simulink model "EBDsimu"  (R2024b)
settings: Solver=VariableStepAuto  StartTime=0.0  StopTime=10  RelTol=1e-3
values from neighbouring files (symbols this model uses):
  dar = 1.5    [EBD.m]
  dav = 1.5    [EBD.m]
  Flim = f*m*g/4    (= 1962)    [ABS.m]    (also in EBD.m)
  g = 9.81    [ABS.m]    (also in EBD.m)
  h = 0.7    [EBD.m]
  J = 0.5    [ABS.m]    (also in EBD.m; TD1_2_3.m = 0.2)
  Kd = 0    [ABS.m]    (also in EBD.m)
  Ki = 20    [ABS.m]    (also in EBD.m = 0)
  Kp = 50    [ABS.m]    (also in EBD.m = 1; TD1_2_3.m = 20)
  L = 3    [EBD.m]    (also in TD1_2_3.m = 0.01216)
  m = 1000    [ABS.m]    (also in EBD.m)
  rRoue = 0.3    [ABS.m]    (also in EBD.m)
  v0 = 27.77    [ABS.m]    (also in EBD.m)
  w0 = v0/rRoue    (= 92.5666666667)    [ABS.m]    (also in EBD.m)
undefined symbols (not defined in the file or in its folder): DiscIntNeverNeededParam
libraries: simulink x9
settings Model: Creator=E306-PC2  LastModifiedBy=clave

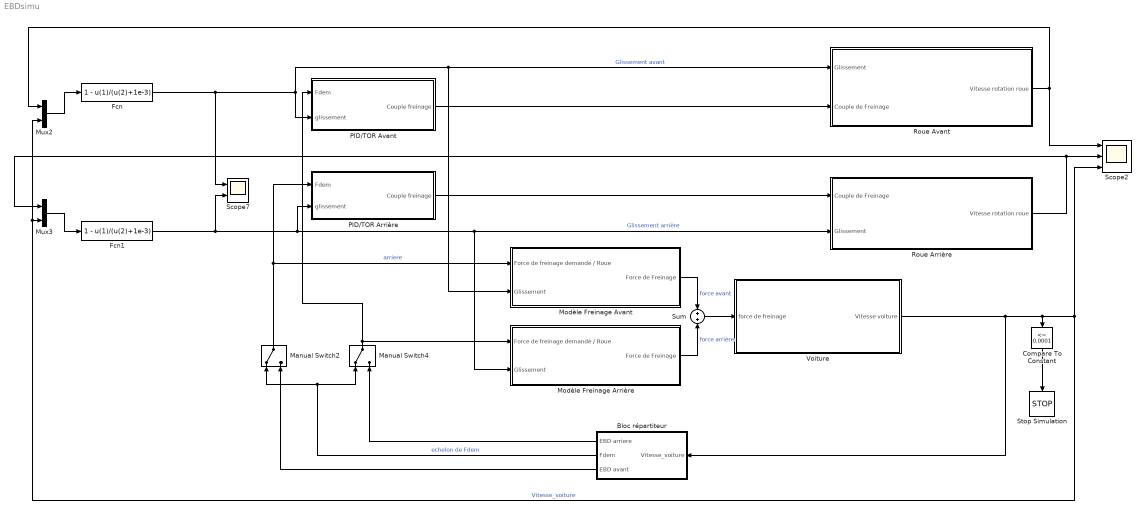
== system EBDsimu ==
  Bloc répartiteur : Subsystem
  Compare To Constant : simulink/Logic and Bit Operations/Compare To Constant  relop=<=  const=0.0001  OutDataTypeStr=boolean
  Fcn : Fcn  Expr=1 - u(1)/(u(2)+1e-3)
  Fcn1 : Fcn  Expr=1 - u(1)/(u(2)+1e-3)
  Manual Switch2 : ManualSwitch
  Manual Switch4 : ManualSwitch
  Modèle Freinage Arrière : Subsystem
  Modèle Freinage Avant : Subsystem
  Mux2 : Mux  Inputs=2
  Mux3 : Mux  Inputs=2
  PID/TOR Arrière : Subsystem
  PID/TOR Avant : Subsystem
  Roue Arrière : Subsystem
  Roue Avant : Subsystem
  Scope2 : Scope  NumInputPorts=3
  Scope7 : Scope  NumInputPorts=2
  Stop Simulation : Stop
  Sum : Sum
  Voiture : Subsystem
  wires:
  Roue Avant/1(Vitesse rotation roue) -> Scope2/1, Mux2/1
  Fcn/1 -> PID/TOR Avant/2(glissement), Roue Avant/1(Glissement), Modèle Freinage Avant/2(Glissement), Scope7/1  "Glissement avant"
  Roue Arrière/1(Vitesse rotation roue) -> Mux3/1, Scope2/2
  Fcn1/1 -> Scope7/2, Modèle Freinage Arrière/2(Glissement), Roue Arrière/2(Glissement), PID/TOR Arrière/2(glissement)  "Glissement arrière"
  Sum/1 -> Voiture/1(force de freinage)
  Mux2/1 -> Fcn/1
  Mux3/1 -> Fcn1/1
  Manual Switch2/1 -> PID/TOR Arrière/1(Fdem), Modèle Freinage Avant/1(Force de freinage demandé / Roue)  "arriere"
  Manual Switch4/1 -> PID/TOR Avant/1(Fdem), Modèle Freinage Arrière/1(Force de freinage demandé / Roue)
  Compare To Constant/1 -> Stop Simulation/1
  Voiture/1(Vitesse voiture) -> Bloc répartiteur/1(Vitesse_voiture), Compare To Constant/1, Scope2/3, Mux2/2, Mux3/2  "Vitesse_voiture"
  PID/TOR Arrière/1(Couple freinage) -> Roue Arrière/1(Couple de Freinage)
  PID/TOR Avant/1(Couple freinage) -> Roue Avant/2(Couple de Freinage)
  Modèle Freinage Avant/1(Force de Freinage) -> Sum/1  "force avant"
  Modèle Freinage Arrière/1(Force de Freinage) -> Sum/2  "force arrière"
  Bloc répartiteur/2(Fdem) -> Manual Switch2/1, Manual Switch4/1  "echelon de Fdem"
  Bloc répartiteur/3(EBD avant) -> Manual Switch2/2
  Bloc répartiteur/1(EBD arriere) -> Manual Switch4/2

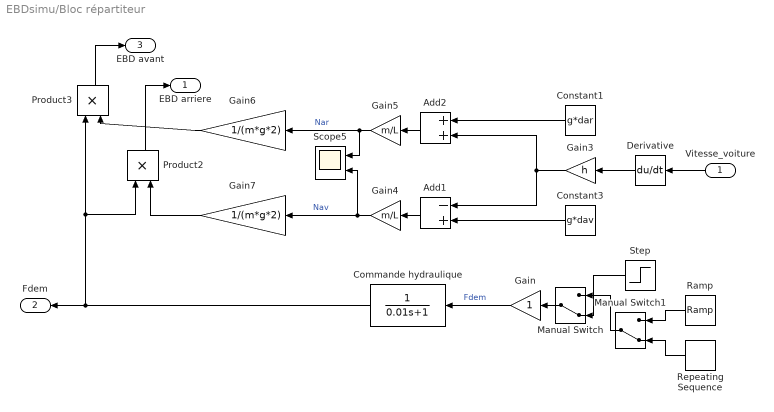
== system EBDsimu/Bloc répartiteur ==
  Vitesse_voiture : Inport
  Add1 : Sum  Inputs=-+
  Add2 : Sum
  Commande hydraulique : TransferFcn  Denominator=[0.01 1]
  Constant1 : Constant  Value=g*dar
  Constant3 : Constant  Value=g*dav
  Derivative : Derivative
  Gain : Gain
  Gain3 : Gain  Gain=h
  Gain4 : Gain  Gain=m/L
  Gain5 : Gain  Gain=m/L
  Gain6 : Gain  Gain=1/(m*g*2)
  Gain7 : Gain  Gain=1/(m*g*2)
  Manual Switch : ManualSwitch  CurrentSetting=0
  Manual Switch1 : ManualSwitch  CurrentSetting=0
  Product2 : Product
  Product3 : Product
  Ramp : simulink/Sources/Ramp  slope=4000  start=0  InitialOutput=0
  Repeating Sequence : simulink/Sources/Repeating Sequence  rep_seq_t=[0 0.5 3 3.5 10]  rep_seq_y=[0 5000 5000 0 0]
  Scope5 : Scope  NumInputPorts=2
  Step : Step  Time=0  After=5000  SampleTime=0
  EBD arriere : Outport
  Fdem : Outport  Port=2
  EBD avant : Outport  Port=3
  wires:
  Repeating Sequence/1 -> Manual Switch1/2
  Add2/1 -> Gain5/1
  Gain4/1 -> Scope5/2, Gain7/1  "Nav"
  Manual Switch1/1 -> Manual Switch/1
  Commande hydraulique/1 -> Fdem/1, Product3/1, Product2/1
  Manual Switch/1 -> Gain/1
  Derivative/1 -> Gain3/1
  Gain3/1 -> Add1/1, Add2/2
  Constant1/1 -> Add2/1
  Gain/1 -> Commande hydraulique/1  "Fdem"
  Gain7/1 -> Product2/2
  Product3/1 -> EBD avant/1
  Add1/1 -> Gain4/1
  Constant3/1 -> Add1/2
  Gain6/1 -> Product3/2
  Product2/1 -> EBD arriere/1
  Gain5/1 -> Scope5/1, Gain6/1  "Nar"
  Step/1 -> Manual Switch/2
  Ramp/1 -> Manual Switch1/1
  Vitesse_voiture/1 -> Derivative/1

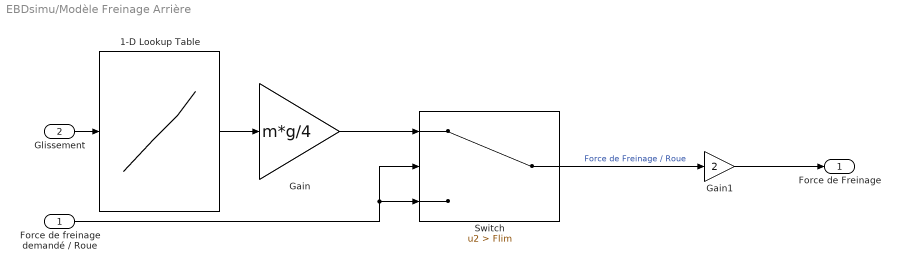
== system EBDsimu/Modèle Freinage Arrière ==
  Force de freinage demandé / Roue : Inport
  Glissement : Inport  Port=2
  1-D Lookup Table : Lookup_n-D  NumberOfTableDimensions=1  BreakpointsForDimension1=[0, 0.1, 0.2, 0.4, 0.6, 0.8, 1]  Table=[0, 0.85, 0.95, 0.75, 0.68, 0.63, 0.6]  InternalRulePriority=Speed  RndMeth=Simplest
  Gain : Gain  Gain=m*g/4
  Gain1 : Gain  Gain=2
  Switch : Switch  Criteria=u2 > Threshold  Threshold=Flim  SaturateOnIntegerOverflow=off  InputSameDT=off
  Force de Freinage : Outport
  wires:
  Gain/1 -> Switch/1
  Force de freinage demandé / Roue/1 -> Switch/3, Switch/2
  Glissement/1 -> 1-D Lookup Table/1
  Switch/1 -> Gain1/1  "Force de Freinage / Roue"
  1-D Lookup Table/1 -> Gain/1
  Gain1/1 -> Force de Freinage/1

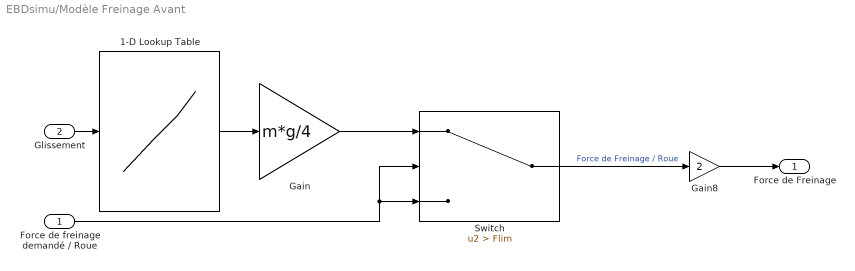
== system EBDsimu/Modèle Freinage Avant ==
  Force de freinage demandé / Roue : Inport
  Glissement : Inport  Port=2
  1-D Lookup Table : Lookup_n-D  NumberOfTableDimensions=1  BreakpointsForDimension1=[0, 0.1, 0.2, 0.4, 0.6, 0.8, 1]  Table=[0, 0.85, 0.95, 0.75, 0.68, 0.63, 0.6]  InternalRulePriority=Speed  RndMeth=Simplest
  Gain : Gain  Gain=m*g/4
  Gain8 : Gain  Gain=2
  Switch : Switch  Criteria=u2 > Threshold  Threshold=Flim  SaturateOnIntegerOverflow=off  InputSameDT=off
  Force de Freinage : Outport
  wires:
  Gain/1 -> Switch/1
  Force de freinage demandé / Roue/1 -> Switch/3, Switch/2
  Glissement/1 -> 1-D Lookup Table/1
  Switch/1 -> Gain8/1  "Force de Freinage / Roue"
  1-D Lookup Table/1 -> Gain/1
  Gain8/1 -> Force de Freinage/1

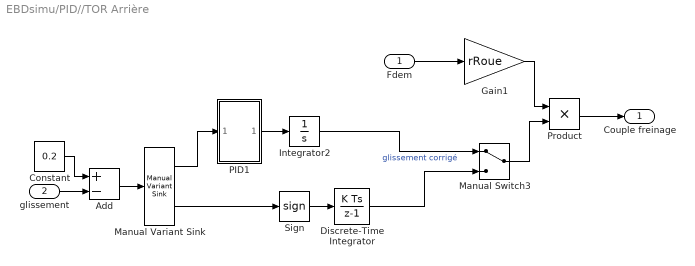
== system EBDsimu/PID//TOR Arrière ==
  Fdem : Inport
  glissement : Inport  Port=2
  Add : Sum  Inputs=+-
  Constant : Constant  Value=0.2
  Discrete-Time Integrator : DiscreteIntegrator  gainval=40  SampleTime=1e-4  LimitOutput=on  UpperSaturationLimit=Flim  ICPrevOutput=DiscIntNeverNeededParam  ICPrevScaledInput=DiscIntNeverNeededParam
  Gain1 : Gain  Gain=rRoue
  Integrator2 : Integrator  LimitOutput=on  UpperSaturationLimit=2000  LowerSaturationLimit=0
  Manual Variant Sink : simulink/Signal Routing/Manual Variant Sink  NumChoices=2  LabelModeActiveChoice=V_1
  Manual Switch3 : ManualSwitch
  PID1 : Subsystem
  Product : Product
  Sign : Signum
  Couple freinage : Outport
  wires:
  Gain1/1 -> Product/1
  Manual Switch3/1 -> Product/2
  Constant/1 -> Add/1
  Add/1 -> Manual Variant Sink/1
  Product/1 -> Couple freinage/1
  Fdem/1 -> Gain1/1
  glissement/1 -> Add/2
  Manual Variant Sink/2 -> Sign/1
  Sign/1 -> Discrete-Time Integrator/1
  Manual Variant Sink/1 -> PID1/1(1)
  Integrator2/1 -> Manual Switch3/1  "glissement corrigé"
  PID1/1(Out1) -> Integrator2/1
  Discrete-Time Integrator/1 -> Manual Switch3/2

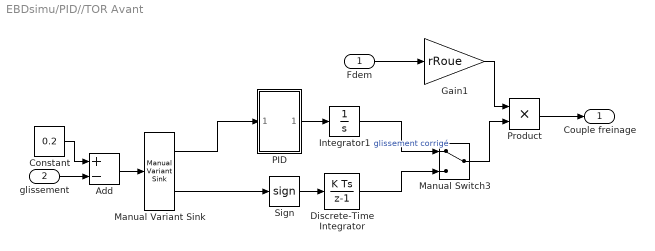
== system EBDsimu/PID//TOR Avant ==
  Fdem : Inport
  glissement : Inport  Port=2
  Add : Sum  Inputs=+-
  Constant : Constant  Value=0.2
  Discrete-Time Integrator : DiscreteIntegrator  gainval=40  SampleTime=1e-4  LimitOutput=on  UpperSaturationLimit=Flim  ICPrevOutput=DiscIntNeverNeededParam  ICPrevScaledInput=DiscIntNeverNeededParam
  Gain1 : Gain  Gain=rRoue
  Integrator1 : Integrator  LimitOutput=on  UpperSaturationLimit=2000  LowerSaturationLimit=0
  Manual Variant Sink : simulink/Signal Routing/Manual Variant Sink  NumChoices=2  LabelModeActiveChoice=V_1
  Manual Switch3 : ManualSwitch
  PID : Subsystem
  Product : Product
  Sign : Signum
  Couple freinage : Outport
  wires:
  Discrete-Time Integrator/1 -> Manual Switch3/2
  Gain1/1 -> Product/1
  Integrator1/1 -> Manual Switch3/1  "glissement corrigé"
  PID/1(Out1) -> Integrator1/1
  Manual Switch3/1 -> Product/2
  Constant/1 -> Add/1
  Product/1 -> Couple freinage/1
  Fdem/1 -> Gain1/1
  glissement/1 -> Add/2
  Manual Variant Sink/2 -> Sign/1
  Sign/1 -> Discrete-Time Integrator/1
  Add/1 -> Manual Variant Sink/1
  Manual Variant Sink/1 -> PID/1(1)

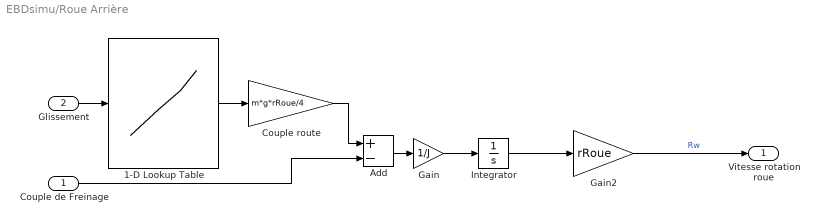
== system EBDsimu/Roue Arrière ==
  Couple de Freinage : Inport
  Glissement : Inport  Port=2
  1-D Lookup Table : Lookup_n-D  NumberOfTableDimensions=1  BreakpointsForDimension1=[0, 0.1, 0.2, 0.4, 0.6, 0.8, 1]  Table=[0, 0.85, 0.95, 0.75, 0.68, 0.63, 0.6]  InternalRulePriority=Speed  RndMeth=Simplest
  Add : Sum  Inputs=+-
  Couple route : Gain  Gain=m*g*rRoue/4
  Gain : Gain  Gain=1/J
  Gain2 : Gain  Gain=rRoue
  Integrator : Integrator  InitialCondition=w0  LimitOutput=on  LowerSaturationLimit=0
  Vitesse rotation roue : Outport
  wires:
  Couple de Freinage/1 -> Add/2
  Couple route/1 -> Add/1
  Glissement/1 -> 1-D Lookup Table/1
  1-D Lookup Table/1 -> Couple route/1
  Gain/1 -> Integrator/1
  Add/1 -> Gain/1
  Integrator/1 -> Gain2/1
  Gain2/1 -> Vitesse rotation roue/1  "Rw"

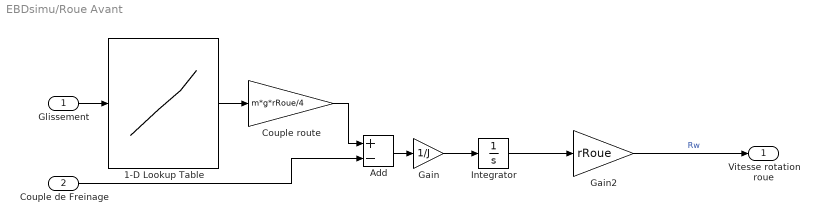
== system EBDsimu/Roue Avant ==
  Glissement : Inport
  Couple de Freinage : Inport  Port=2
  1-D Lookup Table : Lookup_n-D  NumberOfTableDimensions=1  BreakpointsForDimension1=[0, 0.1, 0.2, 0.4, 0.6, 0.8, 1]  Table=[0, 0.85, 0.95, 0.75, 0.68, 0.63, 0.6]  InternalRulePriority=Speed  RndMeth=Simplest
  Add : Sum  Inputs=+-
  Couple route : Gain  Gain=m*g*rRoue/4
  Gain : Gain  Gain=1/J
  Gain2 : Gain  Gain=rRoue
  Integrator : Integrator  InitialCondition=w0  LimitOutput=on  LowerSaturationLimit=0
  Vitesse rotation roue : Outport
  wires:
  Couple de Freinage/1 -> Add/2
  Couple route/1 -> Add/1
  Glissement/1 -> 1-D Lookup Table/1
  1-D Lookup Table/1 -> Couple route/1
  Gain/1 -> Integrator/1
  Add/1 -> Gain/1
  Integrator/1 -> Gain2/1
  Gain2/1 -> Vitesse rotation roue/1  "Rw"

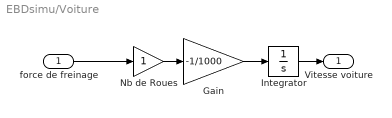
== system EBDsimu/Voiture ==
  force de freinage : Inport
  Gain : Gain  Gain=-1/1000
  Integrator : Integrator  InitialCondition=v0  LimitOutput=on  LowerSaturationLimit=0
  Nb de Roues : Gain
  Vitesse voiture : Outport
  wires:
  Gain/1 -> Integrator/1
  Integrator/1 -> Vitesse voiture/1
  Nb de Roues/1 -> Gain/1
  force de freinage/1 -> Nb de Roues/1

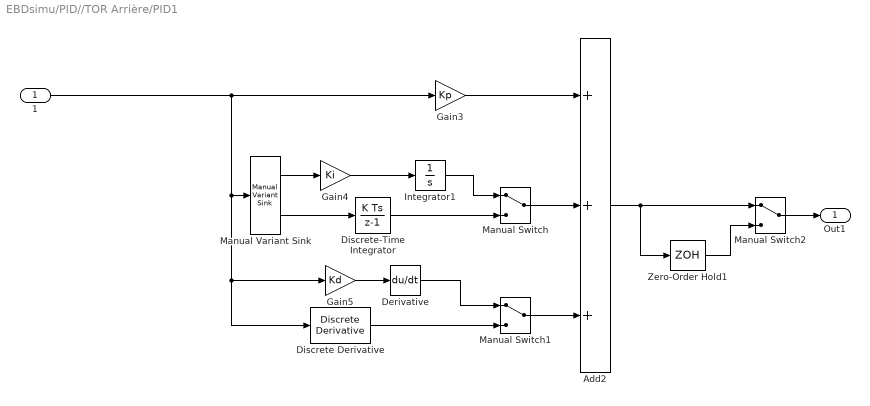
== system EBDsimu/PID//TOR Arrière/PID1 ==
  1 : Inport
  Add2 : Sum  Inputs=+++
  Derivative : Derivative
  Discrete Derivative : simulink/Discrete/Discrete Derivative  gainval=Kd  ICPrevScaledInput=0.0  OutMin=[]  OutMax=[]  OutDataType=fixdt(1, 16)  OutScaling=2^-10  DoSatur=off
  Discrete-Time Integrator : DiscreteIntegrator  gainval=Ki  SampleTime=1e-4  ICPrevOutput=DiscIntNeverNeededParam  ICPrevScaledInput=DiscIntNeverNeededParam
  Gain3 : Gain  Gain=Kp
  Gain4 : Gain  Gain=Ki
  Gain5 : Gain  Gain=Kd
  Integrator1 : Integrator  LimitOutput=on  UpperSaturationLimit=Flim  LowerSaturationLimit=0
  Manual Variant Sink : simulink/Signal Routing/Manual Variant Sink  NumChoices=2  LabelModeActiveChoice=V_1
  Manual Switch : ManualSwitch
  Manual Switch1 : ManualSwitch
  Manual Switch2 : ManualSwitch
  Zero-Order Hold1 : ZeroOrderHold  SampleTime=1e-4
  Out1 : Outport
  wires:
  Gain3/1 -> Add2/1
  Gain4/1 -> Integrator1/1
  Gain5/1 -> Derivative/1
  Manual Switch/1 -> Add2/2
  Integrator1/1 -> Manual Switch/1
  Manual Switch1/1 -> Add2/3
  Derivative/1 -> Manual Switch1/1
  Add2/1 -> Zero-Order Hold1/1, Manual Switch2/1
  Discrete Derivative/1 -> Manual Switch1/2
  1/1 -> Manual Variant Sink/1, Discrete Derivative/1, Gain5/1, Gain3/1
  Discrete-Time Integrator/1 -> Manual Switch/2
  Manual Switch2/1 -> Out1/1
  Zero-Order Hold1/1 -> Manual Switch2/2
  Manual Variant Sink/1 -> Gain4/1
  Manual Variant Sink/2 -> Discrete-Time Integrator/1

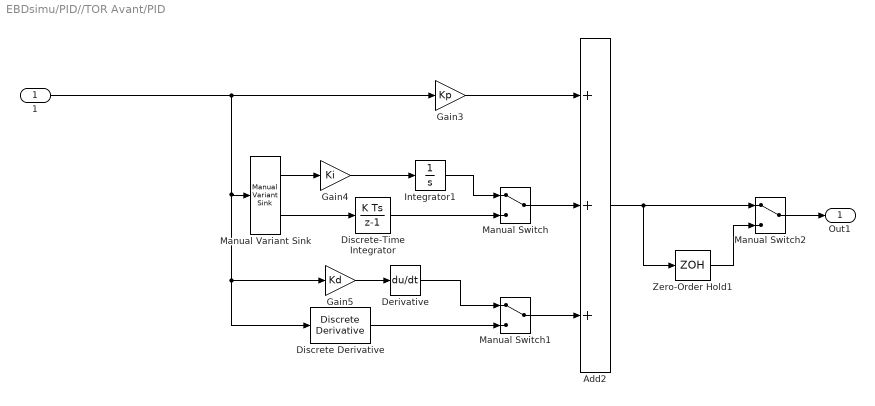
== system EBDsimu/PID//TOR Avant/PID ==
  1 : Inport
  Add2 : Sum  Inputs=+++
  Derivative : Derivative
  Discrete Derivative : simulink/Discrete/Discrete Derivative  gainval=Kd  ICPrevScaledInput=0.0  OutMin=[]  OutMax=[]  OutDataType=fixdt(1, 16)  OutScaling=2^-10  DoSatur=off
  Discrete-Time Integrator : DiscreteIntegrator  gainval=Ki  SampleTime=1e-4  ICPrevOutput=DiscIntNeverNeededParam  ICPrevScaledInput=DiscIntNeverNeededParam
  Gain3 : Gain  Gain=Kp
  Gain4 : Gain  Gain=Ki
  Gain5 : Gain  Gain=Kd
  Integrator1 : Integrator  LimitOutput=on  UpperSaturationLimit=5000  LowerSaturationLimit=0
  Manual Variant Sink : simulink/Signal Routing/Manual Variant Sink  NumChoices=2  LabelModeActiveChoice=V_1
  Manual Switch : ManualSwitch
  Manual Switch1 : ManualSwitch
  Manual Switch2 : ManualSwitch
  Zero-Order Hold1 : ZeroOrderHold  SampleTime=1e-4
  Out1 : Outport
  wires:
  Gain3/1 -> Add2/1
  Gain4/1 -> Integrator1/1
  Gain5/1 -> Derivative/1
  Manual Switch/1 -> Add2/2
  Integrator1/1 -> Manual Switch/1
  Discrete-Time Integrator/1 -> Manual Switch/2
  Manual Switch1/1 -> Add2/3
  Derivative/1 -> Manual Switch1/1
  Discrete Derivative/1 -> Manual Switch1/2
  Add2/1 -> Manual Switch2/1, Zero-Order Hold1/1
  Zero-Order Hold1/1 -> Manual Switch2/2
  Manual Switch2/1 -> Out1/1
  Manual Variant Sink/1 -> Gain4/1
  Manual Variant Sink/2 -> Discrete-Time Integrator/1
  1/1 -> Manual Variant Sink/1, Discrete Derivative/1, Gain5/1, Gain3/1
